simulink model "SMO_lab9"  (R2025b)
settings: Solver=FixedStepDiscrete  StartTime=0.0  StopTime=4000  RelTol=1e-3
values from neighbouring files (symbols this model uses):
  m = 'SMO_lab9'    [lab9.m]
undefined symbols (not defined in the file or in its folder): n
settings Model: Creator=saliy_03jey6u  LastModifiedBy=saliy_03jey6u

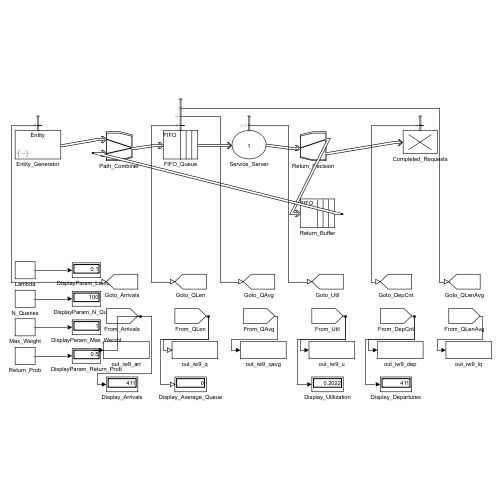
[thumbnail: Simulink's stored preview of the top-level diagram]
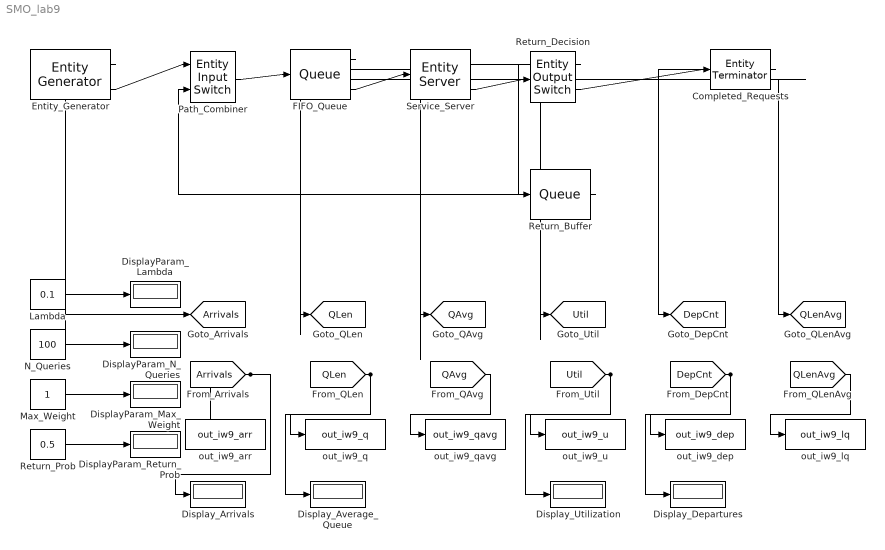
== system SMO_lab9 ==
  Completed_Requests : EntityTerminator  InputPortMessageModes=m  NumberEntitiesArrived=on
      settings: OutputPortMap=o0
  DisplayParam_Lambda : Display
  DisplayParam_Max_Weight : Display
  DisplayParam_N_Queries : Display
  DisplayParam_Return_Prob : Display
  Display_Arrivals : Display
  Display_Average_Queue : Display
  Display_Departures : Display
  Display_Utilization : Display
  Entity_Generator : EntityGenerator  OutputPortMessageModes=n,m  TimeSource=MATLAB action  IntergenerationTimeAction=dt = -log(rand())/0.1;  GenerateAction=st = -log(rand())/1 + rand()*1;  AttributeName=st  NumberEntitiesDeparted=on  EntityType=Structured  EntityTypeName=Entity
      settings: OutputPortMap=o0,o3
  FIFO_Queue : Queue  InputPortMessageModes=m  OutputPortMessageModes=n,n,n,m  Capacity=10  NumberEntitiesInBlock=on  AverageWait=on  AverageQueueLength=on
      settings: OutputPortMap=o1,o2,o3,o5
  Lambda : Constant  Value=0.1
  Max_Weight : Constant
  N_Queries : Constant  Value=100
  Path_Combiner : EntityInputSwitch  InputPortMessageModes=m,m  OutputPortMessageModes=m
  Return_Buffer : Queue  InputPortMessageModes=m  OutputPortMessageModes=m  Capacity=10
  Return_Decision : EntityOutputSwitch  InputPortMessageModes=m  OutputPortMessageModes=m,m  SwitchingCriterion=Equiprobable  SwitchAttributeName=Attribute1
  Return_Prob : Constant  Value=0.5
  Service_Server : EntityServer  InputPortMessageModes=m  OutputPortMessageModes=n,m  Capacity=1  ServiceTimeSource=Attribute  ServiceTimeAttributeName=st  Utilization=on
      settings: OutputPortMap=o5,o9
  out_iw9_arr : ToWorkspace  VariableName=out_iw9_arr  SaveFormat=Timeseries  SampleTime=-1
  out_iw9_dep : ToWorkspace  VariableName=out_iw9_dep  SaveFormat=Timeseries  SampleTime=-1
  out_iw9_lq : ToWorkspace  VariableName=out_iw9_lq  SaveFormat=Timeseries  SampleTime=-1
  out_iw9_q : ToWorkspace  VariableName=out_iw9_q  SaveFormat=Timeseries  SampleTime=-1
  out_iw9_qavg : ToWorkspace  VariableName=out_iw9_qavg  SaveFormat=Timeseries  SampleTime=-1
  out_iw9_u : ToWorkspace  VariableName=out_iw9_u  SaveFormat=Timeseries  SampleTime=-1
  tag scope: Arrivals=global, DepCnt=global, QAvg=global, QLen=global, QLenAvg=global, Util=global
  wires:
  Entity_Generator/2 -> Path_Combiner/1
  Path_Combiner/1 -> FIFO_Queue/1
  FIFO_Queue/4 -> Service_Server/1
  Service_Server/2 -> Return_Decision/1
  Return_Decision/1 -> Return_Buffer/1
  Return_Buffer/1 -> Path_Combiner/2
  Return_Decision/2 -> Completed_Requests/1
  Lambda/1 -> DisplayParam_Lambda/1
  N_Queries/1 -> DisplayParam_N_Queries/1
  Max_Weight/1 -> DisplayParam_Max_Weight/1
  Return_Prob/1 -> DisplayParam_Return_Prob/1
  Entity_Generator/1 -> [Arrivals]
  [Arrivals] -> out_iw9_arr/1, Display_Arrivals/1
  FIFO_Queue/1 -> [QLen]
  [QLen] -> out_iw9_q/1, Display_Average_Queue/1
  FIFO_Queue/2 -> [QAvg]
  [QAvg] -> out_iw9_qavg/1
  FIFO_Queue/3 -> [QLenAvg]
  [QLenAvg] -> out_iw9_lq/1
  Service_Server/1 -> [Util]
  [Util] -> out_iw9_u/1, Display_Utilization/1
  Completed_Requests/1 -> [DepCnt]
  [DepCnt] -> out_iw9_dep/1, Display_Departures/1
